simulink model "LunarMicrogrid_Combined_PVOnly_backup"  (R2026b)
settings: Solver=ode23t  StopTime=simulation.timeSim  MaxStep=1/(5*solarPlant.converterSwitchingFrequency)  AbsTol=1e-3
PreLoadFcn:
  | run('LunarMicrogridA_Data');
undefined symbols (not defined in the file or in its folder): battery, bms, bmsController, boostController, connectedLoad, dcVoltage, lunarCase, maxSoC, maxVdc, minIrrad, minSoC, minVdc, olTime, sensor, solarPanel, solarPlant
libraries: fl_lib x17, nesl_utility x15, simulink x13, ee_lib x6, eePwmGenerator x3, simulink_extras x2, batteryecm_lib x1
(part 1 of 2)
settings Model: Creator=The MathWorks, Inc.  LastModifiedBy=Samiya
settings SolverCC: AutoScaleAbsTol=off
settings DataIOCC: DSMLogging=off  ReturnWorkspaceOutputs=off  SaveOutput=off  SaveTime=off  SignalLoggingName=SolarPVDCWithBattery_logDB
settings OptimizationCC: ReuseModelBlockBuffer=off
settings DebuggingCC: SymbolicDimsDataTypeCodeGenerationDiagnostic=none
settings SFSimCC: CustomCodeUndefinedFunction=UseInterfaceOnly
settings RTWCC: DLArmComputeVersion=19.05
settings SimscapeCC: SimscapeLogName=simlog_SolarPVDCWithBattery  SimscapeLogSimulationStatistics=on  SimscapeLogType=all  SimscapeUseEnergyAccounting=off

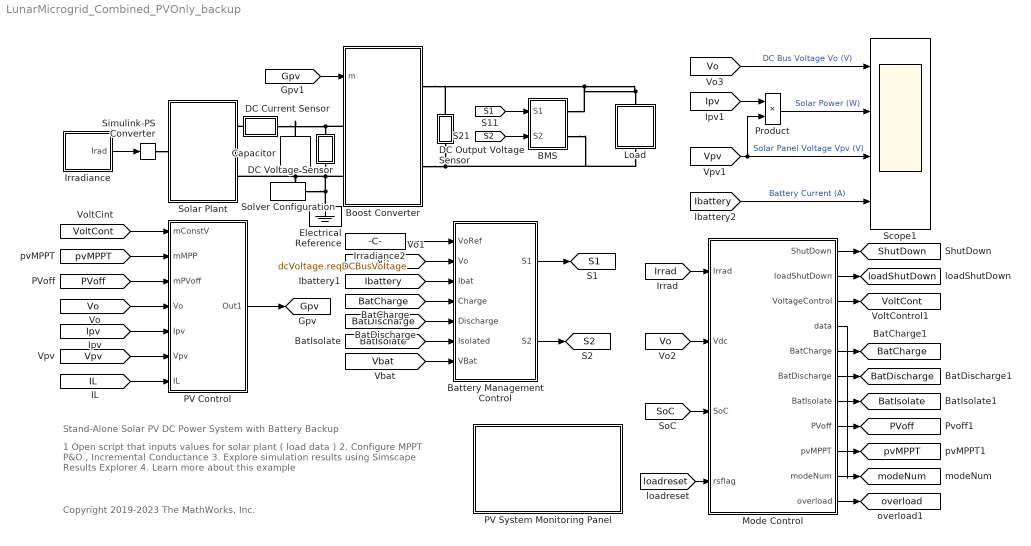
== system LunarMicrogrid_Combined_PVOnly_backup ==
  note: 1 Open script that inputs values for solar plant ( load data )
      | 2. Configure MPPT P&O , Incremental Conductance
      | 3. Explore simulation results using Simscape Results Explorer
      | 4. Learn more about this example
  note: Stand-Alone Solar PV DC Power System with Battery Backup
  note: Copyright 2019-2023 The MathWorks, Inc.
  BMS : Subsystem
  Battery Management Control : Subsystem
  Boost Converter : Subsystem  VariantControl=boostCircuit == 1
  Capacitor : fl_lib/Electrical/Electrical Elements/Capacitor  c=boost.inputCapacitor F  r=1e-6 Ohm  g=0 1/Ohm  i_specify=off  i_priority=None  i=0 A  i_nominal_specify=off  i_nominal_value=1  i_nominal_unit=A  v_specify=off  v_priority=None  v=solarPlant.startMPPTValue V  v_nominal_specify=off  v_nominal_value=1  v_nominal_unit=V  vc_specify=on  vc_priority=High  vc=solarPVInputCapacitorInitialVoltage V  vc_nominal_specify=off  vc_nominal_value=1  vc_nominal_unit=V
  DC Current Sensor : Subsystem
      mask Display: disp('i')
  DC Output Voltage Sensor : Subsystem
      mask Display: disp('v')
  DC Voltage Sensor : Subsystem
      mask Display: disp('v');
  Electrical Reference : fl_lib/Electrical/Electrical Elements/Electrical Reference
  Irradiance : Subsystem
  Irradiance2 : Constant  Value=dcVoltage.reqDCBusVoltage
  Load : Subsystem
  Mode Control : Stateflow chart  TreatAsAtomicUnit=on
  PV Control : Subsystem
  PV System Monitoring Panel : Subsystem
  Product : Product
  Scope1 : Scope  NumInputPorts=4
      settings: TimeSpan=simulation.timeSim  ActiveDisplayYMinimum=-72.27632  ActiveDisplayYMaximum=650.48692
  Simulink-PS Converter : nesl_utility/Simulink-PS Converter  PhysicalDomain=network_engine_domain  SubClassName=ps_input  LeftPortType=input  RightPortType=output  PseudoPeriodic=off  Frequencies=[]  NoiseDistribution=none  NoiseParameters=[]  Unit=1  AffineConversion=off  FilteringAndDerivatives=provide  SimscapeFilterOrder=1  InputFilterTimeConstant=0.001  UdotUserProvided=0
  Solar Plant : Subsystem
  Solver Configuration : nesl_utility/Solver Configuration  PhysicalDomain=network_engine_domain  SubClassName=solver  LeftPortType=input  RightPortType=generic  Tones=[]  Harmonics=[]  SimulateNoise=off  Profile=off  UseLocalSampling=off  EnableSwitchedLinearOptims=on  FrequencyDomain=off  UseCCode=off  RelTol=0.001  AbsTol=1e-06  MinStep=1e-09  ToWorkspace=off  RevertToSquareIcSolve=off  NumHomotopyIterations=100  PhasorMode=off  PhasorModeNumHarmonics=1  ConsistencySolver=NEWTON_FTOL  CanonicalOrdering=UNORDERED  OptimizeIntermediates=UNOPTIMIZED  MulticoreSolverChoice=BACKWARD_EULER  IndexReductionMethod=DerivativeReplacement  DoDC=off  ResidualTolerance=1e-9  ConsistencyTolSource=GLOBAL  ConsistencyAbsTol=0.001  ConsistencyRelTol=0.001  ConsistencyTolFactor=0.001  UseLocalSolver=off  LocalSolverChoice=NE_TRAPEZOIDAL_ADVANCER  ResolveIndetEquations=on  FunctionEvalNumThread=1  LocalSolverSampleTime=2e-6  DoFixedCost=off  MaxNonlinIter=10  MaxModeIter=2  ComputeImpulses=off  ImpulseIterations=2  LinearAlgebra=auto  LinearAlgebraNumThread=0  EquationFormulation=NE_TIME_EF  DelaysMemoryBudget=1024  AutomaticFiltering=on  FilteringTimeConstant=0.001  PartitionStorageMethod=AS_NEEDED  PartitionMemoryBudget=1024  PartitionMethod=FAST  MultibodyUseLocalSolver=off  MultibodyLocalSolverChoice=ODE1  MultibodyLocalSolverSampleTime=0.001
  tag scope: BatCharge=global, BatDischarge=global, BatIsolate=global, Gpv=global, PVoff=global, S1=global, S2=global, ShutDown=global, VoltCont=global, loadShutDown=global, modeNum=global, overload=global, pvMPPT=global
  wires:
  Mode Control/6(BatDischarge) -> [BatDischarge]
  [Vpv] -> Scope1/3, Product/2  "Solar Panel Voltage Vpv (V)"
  Battery Management Control/2(S2) -> [S2]
  [Ibattery] -> Battery Management Control/3(Ibat)
  Product/1 -> Scope1/2  "Solar Power (W)"
  [Vbat] -> Battery Management Control/7(VBat)
  [Ipv] -> PV Control/5(Ipv)
  Irradiance/1(Irad) -> Simulink-PS Converter/1
  [IL] -> PV Control/7(IL)
  Mode Control/2(loadShutDown) -> [loadShutDown]
  Mode Control/10(modeNum) -> [modeNum]
  [BatDischarge] -> Battery Management Control/5(Discharge)
  Mode Control/11(overload) -> [overload]
  [Ipv] -> Product/1
  [PVoff] -> PV Control/3(mPVoff)
  Mode Control/1(ShutDown) -> [ShutDown]
  Mode Control/3(VoltageControl) -> [VoltCont]
  [BatIsolate] -> Battery Management Control/6(Isolated)
  [Vo] -> Mode Control/2(Vdc)
  [pvMPPT] -> PV Control/2(mMPP)
  Mode Control/9(pvMPPT) -> [pvMPPT]
  [loadreset] -> Mode Control/4(rsflag)
  [SoC] -> Mode Control/3(SoC)
  Mode Control/7(BatIsolate) -> [BatIsolate]
  [Gpv] -> Boost Converter/1(m)
  PV Control/1(Out1) -> [Gpv]
  Irradiance2/1 -> Battery Management Control/1(VoRef)
  [VoltCont] -> PV Control/1(mConstV)
  [Irrad] -> Mode Control/1(Irrad)
  Mode Control/8(PVoff) -> [PVoff]
  [Vo] -> Scope1/1  "DC Bus Voltage Vo (V)"
  Mode Control/5(BatCharge) -> [BatCharge]
  Battery Management Control/1(S1) -> [S1]
  [Ibattery] -> Scope1/4  "Battery Current (A)"
  [Vo] -> PV Control/4(Vo)
  [Vo] -> Battery Management Control/2(Vo)
  [S2] -> BMS/2(S2)
  [Vpv] -> PV Control/6(Vpv)
  [BatCharge] -> Battery Management Control/4(Charge)
  [S1] -> BMS/1(S1)
  Mode Control/4(data) -> ?
  connections:
  Load/LConn1 -- BMS/RConn1 -- Boost Converter/RConn1 -- DC Output Voltage Sensor/RConn1
  Boost Converter/RConn2 -- BMS/RConn2 -- Load/RConn1 -- DC Output Voltage Sensor/LConn1
  Solver Configuration/RConn1 -- Solar Plant/RConn2 -- Capacitor/RConn1 -- Boost Converter/LConn2 -- DC Voltage Sensor/LConn1 -- Electrical Reference/LConn1
  Boost Converter/LConn1 -- DC Voltage Sensor/RConn1 -- DC Current Sensor/LConn1 -- Capacitor/LConn1
  DC Current Sensor/RConn1 -- Solar Plant/RConn1
  Simulink-PS Converter/RConn1 -- Solar Plant/LConn1

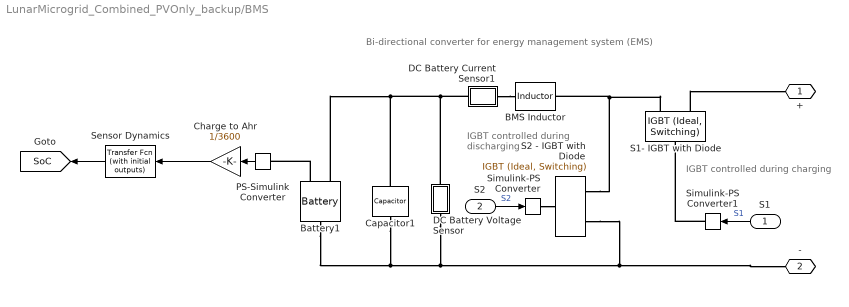
== system LunarMicrogrid_Combined_PVOnly_backup/BMS ==
  note: IGBT controlled during charging
  note: Bi-directional converter for energy management system (EMS)
  note: IGBT controlled during discharging
  S1 : Inport
  S2 : Inport  Port=2
  BMS Inductor : fl_lib/Electrical/Electrical Elements/Inductor  l=bms.batteryChargingInductor H  r=bms.batteryChargingInductorResistance Ohm  g=1e-9 1/Ohm  i_specify=off  i_priority=High  i=0 A  i_nominal_specify=off  i_nominal_value=1  i_nominal_unit=A  v_specify=off  v_priority=High  v=0 V  v_nominal_specify=off  v_nominal_value=1  v_nominal_unit=V  i_L_specify=on  i_L_priority=High  i_L=0 A  i_L_nominal_specify=off  i_L_nominal_value=1  i_L_nominal_unit=A
      settings: LogSimulationData=on
  Battery1 : batteryecm_lib/Battery  Vnom=battery.nominalBatteryVoltage V  prm_dir=1  R1_dis=2 Ohm  R1_ch=2 Ohm  R1=0.01 Ohm  prm_AH=2  AH=connectedLoad.batteryAmpHr hr*A  V1=battery.minBatteryNominalVoltage V  AH1=connectedLoad.batteryAmpHr*0.2 hr*A  prm_R2=2  R2=2000 Ohm  Tmeas=298.15 K  charge_measurement_port=simscape.enum.battery.enable.yes  prm_dyn=1  Rp1=0.005 Ohm  tau1=30 s  Rp2=0.005 Ohm  tau2=30 s  Rp3=0.005 Ohm  tau3=30 s  Rp4=0.005 Ohm  tau4=30 s  Rp5=0.005 Ohm  tau5=30 s  prm_fade=1  N_fade=100  AH_fade=45 hr*A  R1_fade=2.02 Ohm  R1_ch_fade=2.02 Ohm  V1_fade=10.35 V  prm_age=1  prm_age_OCV=1  OCV_age=0.9  SOC_age=60  Tmeas_age=298.15 K  delta_time_age_vec=[0] d  temperature_age_vec=[273] K  OCV_scaling_age=2.2134e6  OCV_offset_age=1.632e6  temp_exp_age=0.515833569 V  t_exp_age=0.75  Vnom_T2=12 V  R1_T2=2.2 Ohm  R1_T2_dis=2.2 Ohm  R1_T2_ch=2.2 Ohm  V1_T2=11.4 V  R2_T2=2200 Ohm  Rp1_T2=0.005 Ohm  tau1_T2=30 s  Rp2_T2=0.005 Ohm  tau2_T2=30 s  Rp3_T2=0.005 Ohm  tau3_T2=30 s  Rp4_T2=0.005 Ohm  tau4_T2=30 s  Rp5_T2=0.005 Ohm  tau5_T2=30 s  Tmeas2=273.15 K  thermal_port=simscape.enum.thermaleffects.omit  thermal_mass=30000 J/K  i_specify=off  i_priority=None  i=0 A  i_nominal_specify=off  i_nominal_value=1  i_nominal_unit=A  v_specify=off  v_priority=None  v=0 V  v_nominal_specify=off  v_nominal_value=1  v_nominal_unit=V  charge_specify=on  charge_priority=High  charge=batteryInitialStateOfCharge hr*A  charge_nominal_specify=off  charge_nominal_value=1  charge_nominal_unit=A*hr  num_cycles_specify=off  num_cycles_priority=High  num_cycles=0  num_cycles_nominal_specify=off  num_cycles_nominal_value=1  num_cycles_nominal_unit=1  temperature_specify=off  temperature_priority=High  temperature=298.15 K  temperature_nominal_specify=off  temperature_nominal_value=1  temperature_nominal_unit=K
  Capacitor1 : fl_lib/Electrical/Electrical Elements/Capacitor  c=boost.outputCapacitor F  r=1e-6 Ohm  g=0 1/Ohm  i_specify=off  i_priority=None  i=0 A  i_nominal_specify=off  i_nominal_value=1  i_nominal_unit=A  v_specify=off  v_priority=None  v=0 V  v_nominal_specify=off  v_nominal_value=1  v_nominal_unit=V  vc_specify=on  vc_priority=High  vc=batteryInputCapacitorInitialVoltage V  vc_nominal_specify=off  vc_nominal_value=1  vc_nominal_unit=V
  Charge to Ahr : Gain  Gain=1/3600
  DC Battery Current Sensor1 : Subsystem
      mask Display: disp('i');
  DC Battery Voltage Sensor : Subsystem
      mask Display: disp('v');
  PS-Simulink Converter : nesl_utility/PS-Simulink Converter  PhysicalDomain=network_engine_domain  SubClassName=ps_output  LeftPortType=input  RightPortType=output  PseudoPeriodic=off  Frequencies=[]  VectorFormat=1-D array  Unit=inherit  AffineConversion=off
  S1- IGBT with Diode : ee_lib/Semiconductors & Converters/IGBT (Ideal, Switching)  port_option=ee.enum.controlport.ps  Vf=0.1 V  Ron=0.001 Ohm  Goff=1e-5 1/Ohm  Vth=2.5 V  diode_param=2  diode_Vf=0.1 V  diode_Ron=0.001 Ohm  diode_Goff=1e-5 1/Ohm  diode_C=50e-9 F  diode_iRM=-235 A  diode_iF=300 A  diode_idot=-50 A/us  diode_trr_param=1  diode_trr_factor=3  diode_trr=15 us  diode_Qrr=1500 s*uA  ice_specify=off  ice_priority=None  ice=0 A  ice_nominal_specify=off  ice_nominal_value=1  ice_nominal_unit=A  vce_specify=off  vce_priority=None  vce=0 V  vce_nominal_specify=off  vce_nominal_value=1  vce_nominal_unit=V  vge_specify=off  vge_priority=None  vge=0 V  vge_nominal_specify=off  vge_nominal_value=1  vge_nominal_unit=V  thermal_loss_option=ee.enum.converters.thermalLossOption.constantvalues  Von_data=[0, .1, .6, .8, 1, 1.3, 1.6, 2, 2.4; 0, .1, .7, 1, 1.2, 1.5, 1.9, 2.4, 2.8] V  Tj=[298.15, 398.15] K  Iout_data=[0, .1, 1, 5, 10, 20, 40, 70, 100] A  tabulateWithVce=false  Eon_data=[0, .0024, .024, .12, .2, .48, 1.04, 2.16, 3.24; 0, .003, .03, .15, .25, .6, 1.3, 2.7, 4.05] * 1e-3 J  Eoff_data=[0, .0007, .0066, .033, .066, .17, .33, .83, 1.5; 0, .001, .01, .05, .1, .25, .5, 1.2, 2.2] * 1e-3 J  Eon_data_3D=[zeros(2, 9, 3)] J  Eoff_data_3D=[zeros(2, 9, 3)] J  Tj_loss=[298.15, 398.15] K  Iout_data_loss=[0, .1, 1, 5, 10, 20, 40, 70, 100] A  Vce_loss=[0, 150, 300] V  Eon_scalar=22.86e-3 J  Eoff_scalar=17.14e-3 J  Voff=300 V  Iout_scalar=600 A  useCurrentFromPreviousCycle=true  currentMeasDelay=0 s  useVoltageFromPreviousCycle=true  voltageMeasDelay=0 s  diodeModelType=ee.enum.converters.diodeModelType.pwl  diodeTableType=ee.enum.diode.tableType.IfMat  diode_ReverseIVType=ee.enum.diode.diodeReverseIV.constant  diode_IfMat=[.07, .12, .19, 1.75, 4.24, 7.32, 11.2; .16, .3, .72, 2.14, 4.02, 6.35, 9.12] A  diode_VfMat=[.9, 1.15, 1.25, 1.5, 1.75, 2.17, 2.6, 2.85; .58, .68, .75, 1.1, 1.38, 1.77, 2.27, 2.7] V  diode_TjVec=[25, 125] degC  diode_VfVec=[.5, .7, .9, 1.3, 1.7, 2.1, 2.5] V  diode_IfVec=[.1, .2, .5, 1, 2, 4, 7, 10] A  diode_IrMat=[1e-06, 2e-06, 5e-06, 1e-05, 2.5e-05, 5e-05, .0001; 2e-06, 5e-06, 1e-05, 4e-05, 8e-05, .0002, .0005] A  diode_VrMat=[10, 100, 200, 250, 300, 325, 350; 10, 70, 160, 220, 270, 300, 320] V  diode_VrVec=[10, 20, 40, 50, 70, 80, 100] V  diode_IrVec=[1e-06, 2e-06, 5e-06, 1e-05, 2e-05, 5e-05, .0001] A  diode_Vr=-600 V  diode_Ls=150 nH  diode_Erec=0.03 J  diode_rec_loss_model=ee.enum.diode.reverseRecoveryModelTabulateUpTo3D.fixed  diode_ErecVal=0 J  diode_scaleWithIandV=true  diode_ErecMat=zeros(2, 3) J  diodeErecMat3D=zeros(2, 3, 2) J  diode_TjrecVec=[298.15, 398.15] K  diode_IfrecVec=[.1, 1, 10] A  diodeVrecVec=[0, 100] V  diode_IrecVal=10 A  diode_VrecVal=10 V  diode_tFilter=1 / 1000 / 100 s  separateThermalPortForDiode=false  thermal_network_parameterization=ee.enum.thermalNetworkTopology.external  Rth=[.08, .5] K/W  Rth_Cauer=[.08, .1, .5] K/W  Rth_Foster=[.08, .14, .22, .16] K/W  thermal_mass_parameterization=ee.enum.thermalNetwork.timeconstant  thermal_mass=[.01, .5] J/K  thermal_mass_Cauer=[.01, .1, .5] J/K  thermal_mass_Foster=[.001, .005, .05, .5] J/K  thermal_time_constant=[.001, .2] s  thermal_time_constant_Cauer=[.001, .1, .2] s  thermal_time_constant_Foster=[7e-05, .0007, .01, .08] s  thermal_mass_initial_temperatures=[25, 25] degC  thermal_mass_initial_temperatures_Cauer=[25, 25, 25] degC  junction_thermal_mass=0.01 J/K  Tvec_initial_Foster=[25, 25, 25, 25] degC  RthDiode=[.03, .2] K/W  RthCauerDiode=[.03, .1, .2] K/W  RthFosterDiode=[.03, .2] K/W  thermalMassDiode=[3, 25] J/K  thermalMassCauerDiode=[3, 10, 25] J/K  thermalMassFosterDiode=[33, 50] J/K  thermalTauDiode=[.1, 5] s  thermalTauCauerDiode=[.1, 1, 5] s  thermalTauFosterDiode=[1, 10] s  thermalMassInitTempDiode=[25, 25] degC  thermalMassInitTempCauerDiode=[25, 25, 25] degC  junctionthermalMassDiode=0.1 J/K  TVecInitialFosterDiode=[25, 25] degC  no_thermal_network=0  IGBT_junction_temperature_specify=off  IGBT_junction_temperature_priority=None  IGBT_junction_temperature=25 degC  IGBT_junction_temperature_nominal_specify=off  IGBT_junction_temperature_nominal_value=1  IGBT_junction_temperature_nominal_unit=degC  diode_junction_temperature_specify=off  diode_junction_temperature_priority=None  diode_junction_temperature=25 degC  diode_junction_temperature_nominal_specify=off  diode_junction_temperature_nominal_value=1  diode_junction_temperature_nominal_unit=degC  Qj_specify=off  Qj_priority=None  Qj=0 W  Qj_nominal_specify=off  Qj_nominal_value=1  Qj_nominal_unit=W  accumulatedSwitchingLosses_specify=off  accumulatedSwitchingLosses_priority=None  accumulatedSwitchingLosses=0 J
  S2 - IGBT with Diode : ee_lib/Semiconductors & Converters/IGBT (Ideal, Switching)  port_option=ee.enum.controlport.ps  Vf=0.1 V  Ron=0.001 Ohm  Goff=1e-5 1/Ohm  Vth=2.5 V  diode_param=2  diode_Vf=0.1 V  diode_Ron=0.001 Ohm  diode_Goff=1e-5 1/Ohm  diode_C=50e-9 F  diode_iRM=-235 A  diode_iF=300 A  diode_idot=-50 A/us  diode_trr_param=1  diode_trr_factor=3  diode_trr=15 us  diode_Qrr=1500 s*uA  ice_specify=off  ice_priority=None  ice=0 A  ice_nominal_specify=off  ice_nominal_value=1  ice_nominal_unit=A  vce_specify=off  vce_priority=None  vce=0 V  vce_nominal_specify=off  vce_nominal_value=1  vce_nominal_unit=V  vge_specify=off  vge_priority=None  vge=0 V  vge_nominal_specify=off  vge_nominal_value=1  vge_nominal_unit=V  thermal_loss_option=ee.enum.converters.thermalLossOption.constantvalues  Von_data=[0, .1, .6, .8, 1, 1.3, 1.6, 2, 2.4; 0, .1, .7, 1, 1.2, 1.5, 1.9, 2.4, 2.8] V  Tj=[298.15, 398.15] K  Iout_data=[0, .1, 1, 5, 10, 20, 40, 70, 100] A  tabulateWithVce=false  Eon_data=[0, .0024, .024, .12, .2, .48, 1.04, 2.16, 3.24; 0, .003, .03, .15, .25, .6, 1.3, 2.7, 4.05] * 1e-3 J  Eoff_data=[0, .0007, .0066, .033, .066, .17, .33, .83, 1.5; 0, .001, .01, .05, .1, .25, .5, 1.2, 2.2] * 1e-3 J  Eon_data_3D=[zeros(2, 9, 3)] J  Eoff_data_3D=[zeros(2, 9, 3)] J  Tj_loss=[298.15, 398.15] K  Iout_data_loss=[0, .1, 1, 5, 10, 20, 40, 70, 100] A  Vce_loss=[0, 150, 300] V  Eon_scalar=22.86e-3 J  Eoff_scalar=17.14e-3 J  Voff=300 V  Iout_scalar=600 A  useCurrentFromPreviousCycle=true  currentMeasDelay=0 s  useVoltageFromPreviousCycle=true  voltageMeasDelay=0 s  diodeModelType=ee.enum.converters.diodeModelType.pwl  diodeTableType=ee.enum.diode.tableType.IfMat  diode_ReverseIVType=ee.enum.diode.diodeReverseIV.constant  diode_IfMat=[.07, .12, .19, 1.75, 4.24, 7.32, 11.2; .16, .3, .72, 2.14, 4.02, 6.35, 9.12] A  diode_VfMat=[.9, 1.15, 1.25, 1.5, 1.75, 2.17, 2.6, 2.85; .58, .68, .75, 1.1, 1.38, 1.77, 2.27, 2.7] V  diode_TjVec=[25, 125] degC  diode_VfVec=[.5, .7, .9, 1.3, 1.7, 2.1, 2.5] V  diode_IfVec=[.1, .2, .5, 1, 2, 4, 7, 10] A  diode_IrMat=[1e-06, 2e-06, 5e-06, 1e-05, 2.5e-05, 5e-05, .0001; 2e-06, 5e-06, 1e-05, 4e-05, 8e-05, .0002, .0005] A  diode_VrMat=[10, 100, 200, 250, 300, 325, 350; 10, 70, 160, 220, 270, 300, 320] V  diode_VrVec=[10, 20, 40, 50, 70, 80, 100] V  diode_IrVec=[1e-06, 2e-06, 5e-06, 1e-05, 2e-05, 5e-05, .0001] A  diode_Vr=-600 V  diode_Ls=150 nH  diode_Erec=0.03 J  diode_rec_loss_model=ee.enum.diode.reverseRecoveryModelTabulateUpTo3D.fixed  diode_ErecVal=0 J  diode_scaleWithIandV=true  diode_ErecMat=zeros(2, 3) J  diodeErecMat3D=zeros(2, 3, 2) J  diode_TjrecVec=[298.15, 398.15] K  diode_IfrecVec=[.1, 1, 10] A  diodeVrecVec=[0, 100] V  diode_IrecVal=10 A  diode_VrecVal=10 V  diode_tFilter=1 / 1000 / 100 s  separateThermalPortForDiode=false  thermal_network_parameterization=ee.enum.thermalNetworkTopology.external  Rth=[.08, .5] K/W  Rth_Cauer=[.08, .1, .5] K/W  Rth_Foster=[.08, .14, .22, .16] K/W  thermal_mass_parameterization=ee.enum.thermalNetwork.timeconstant  thermal_mass=[.01, .5] J/K  thermal_mass_Cauer=[.01, .1, .5] J/K  thermal_mass_Foster=[.001, .005, .05, .5] J/K  thermal_time_constant=[.001, .2] s  thermal_time_constant_Cauer=[.001, .1, .2] s  thermal_time_constant_Foster=[7e-05, .0007, .01, .08] s  thermal_mass_initial_temperatures=[25, 25] degC  thermal_mass_initial_temperatures_Cauer=[25, 25, 25] degC  junction_thermal_mass=0.01 J/K  Tvec_initial_Foster=[25, 25, 25, 25] degC  RthDiode=[.03, .2] K/W  RthCauerDiode=[.03, .1, .2] K/W  RthFosterDiode=[.03, .2] K/W  thermalMassDiode=[3, 25] J/K  thermalMassCauerDiode=[3, 10, 25] J/K  thermalMassFosterDiode=[33, 50] J/K  thermalTauDiode=[.1, 5] s  thermalTauCauerDiode=[.1, 1, 5] s  thermalTauFosterDiode=[1, 10] s  thermalMassInitTempDiode=[25, 25] degC  thermalMassInitTempCauerDiode=[25, 25, 25] degC  junctionthermalMassDiode=0.1 J/K  TVecInitialFosterDiode=[25, 25] degC  no_thermal_network=0  IGBT_junction_temperature_specify=off  IGBT_junction_temperature_priority=None  IGBT_junction_temperature=25 degC  IGBT_junction_temperature_nominal_specify=off  IGBT_junction_temperature_nominal_value=1  IGBT_junction_temperature_nominal_unit=degC  diode_junction_temperature_specify=off  diode_junction_temperature_priority=None  diode_junction_temperature=25 degC  diode_junction_temperature_nominal_specify=off  diode_junction_temperature_nominal_value=1  diode_junction_temperature_nominal_unit=degC  Qj_specify=off  Qj_priority=None  Qj=0 W  Qj_nominal_specify=off  Qj_nominal_value=1  Qj_nominal_unit=W  accumulatedSwitchingLosses_specify=off  accumulatedSwitchingLosses_priority=None  accumulatedSwitchingLosses=0 J
  Sensor Dynamics : simulink_extras/Additional Linear/Transfer Fcn (with initial outputs)  N=[1]  D=[1/sensor.samplingFreq 1]  Y0=minSoC  U0=0
  Simulink-PS Converter : nesl_utility/Simulink-PS Converter  PhysicalDomain=network_engine_domain  SubClassName=ps_input  LeftPortType=input  RightPortType=output  PseudoPeriodic=off  Frequencies=[]  NoiseDistribution=none  NoiseParameters=[]  Unit=1  AffineConversion=off  FilteringAndDerivatives=provide  SimscapeFilterOrder=1  InputFilterTimeConstant=0.001  UdotUserProvided=0
  Simulink-PS Converter1 : nesl_utility/Simulink-PS Converter  PhysicalDomain=network_engine_domain  SubClassName=ps_input  LeftPortType=input  RightPortType=output  PseudoPeriodic=off  Frequencies=[]  NoiseDistribution=none  NoiseParameters=[]  Unit=1  AffineConversion=off  FilteringAndDerivatives=provide  SimscapeFilterOrder=1  InputFilterTimeConstant=0.001  UdotUserProvided=0
  + : PMIOPort  Side=Right
  - : PMIOPort  Port=2  Side=Right
  tag scope: SoC=global
  wires:
  S2/1 -> Simulink-PS Converter/1  "S2"
  S1/1 -> Simulink-PS Converter1/1  "S1"
  PS-Simulink Converter/1 -> Charge to Ahr/1
  Sensor Dynamics/1 -> [SoC]
  Charge to Ahr/1 -> Sensor Dynamics/1
  connections:
  S2 - IGBT with Diode/RConn2 -- Battery1/RConn1 -- Capacitor1/RConn1 -- DC Battery Voltage Sensor/LConn1 -- -/RConn1
  S2 - IGBT with Diode/RConn1 -- S1- IGBT with Diode/RConn2 -- BMS Inductor/RConn1
  S1- IGBT with Diode/RConn1 -- +/RConn1
  Simulink-PS Converter/RConn1 -- S2 - IGBT with Diode/LConn1
  Battery1/LConn2 -- PS-Simulink Converter/LConn1
  Simulink-PS Converter1/RConn1 -- S1- IGBT with Diode/LConn1
  DC Battery Current Sensor1/RConn1 -- BMS Inductor/LConn1
  DC Battery Current Sensor1/LConn1 -- DC Battery Voltage Sensor/RConn1 -- Battery1/LConn1 -- Capacitor1/LConn1

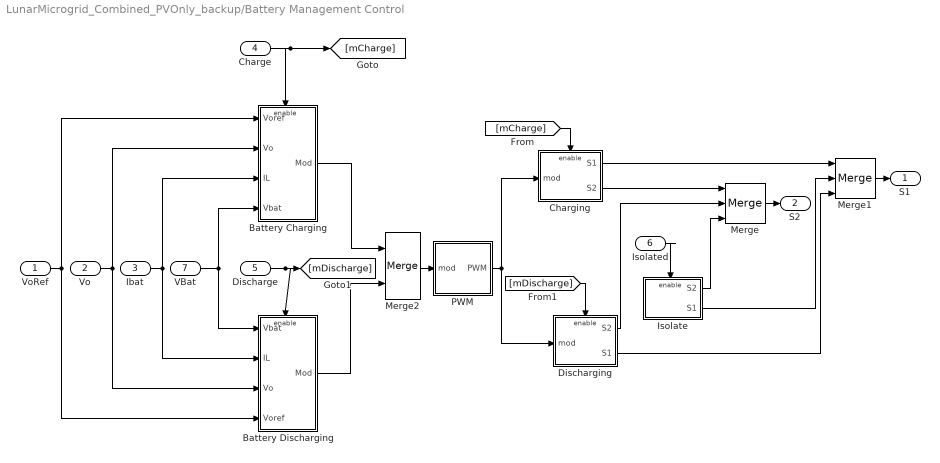
== system LunarMicrogrid_Combined_PVOnly_backup/Battery Management Control ==
  VoRef : Inport
  Vo : Inport  Port=2
  Ibat : Inport  Port=3
  Charge : Inport  Port=4
  Discharge : Inport  Port=5
  Isolated : Inport  Port=6
  VBat : Inport  Port=7
  Battery Charging : Subsystem
  Battery Discharging : Subsystem
  Charging : Subsystem  TreatAsAtomicUnit=on
  Discharging : Subsystem  TreatAsAtomicUnit=on
  Isolate : Subsystem  TreatAsAtomicUnit=on
  Merge : Merge  Inputs=3
  Merge1 : Merge  Inputs=3
  Merge2 : Merge
  PWM : Subsystem
  S1 : Outport
  S2 : Outport  Port=2
  wires:
  Charging/2(S2) -> Merge/1
  Discharging/1(S2) -> Merge/2
  Charging/1(S1) -> Merge1/1
  Isolate/1(S2) -> Merge/3
  Isolate/2(S1) -> Merge1/2
  Discharging/2(S1) -> Merge1/3
  Merge1/1 -> S1/1
  Isolated/1 -> Isolate/Enable
  Vo/1 -> Battery Charging/2(Vo), Battery Discharging/3(Vo)
  Ibat/1 -> Battery Charging/3(IL), Battery Discharging/2(IL)
  Battery Charging/1(Mod) -> Merge2/1
  Battery Discharging/1(Mod) -> Merge2/2
  Merge/1 -> S2/1
  Charge/1 -> [mCharge], Battery Charging/Enable
  Discharge/1 -> Battery Discharging/Enable, [mDischarge]
  [mCharge] -> Charging/Enable
  [mDischarge] -> Discharging/Enable
  PWM/1(PWM) -> Charging/1(mod), Discharging/1(mod)
  Merge2/1 -> PWM/1(mod)
  VoRef/1 -> Battery Charging/1(Voref), Battery Discharging/4(Voref)
  VBat/1 -> Battery Discharging/1(Vbat), Battery Charging/4(Vbat)

== system LunarMicrogrid_Combined_PVOnly_backup/Boost Converter ==
  m : Inport
  AC Current Sensor1 : Subsystem
      mask Display: disp('i');
  DC Bus Capacitor : fl_lib/Electrical/Electrical Elements/Capacitor  c=boost.outputCapacitor F  r=1e-6 Ohm  g=0 1/Ohm  i_specify=off  i_priority=None  i=0 A  i_nominal_specify=off  i_nominal_value=1  i_nominal_unit=A  v_specify=off  v_priority=None  v=0 V  v_nominal_specify=off  v_nominal_value=1  v_nominal_unit=V  vc_specify=on  vc_priority=High  vc=boostOutputCapacitorInitialVoltage V  vc_nominal_specify=off  vc_nominal_value=1  vc_nominal_unit=V
  Diode : fl_lib/Electrical/Electrical Elements/Diode  Vf=0.6 V  Ron=0.3 Ohm  Goff=1e-8 1/Ohm  i_specify=off  i_priority=None  i=0 A  i_nominal_specify=off  i_nominal_value=1  i_nominal_unit=A  v_specify=off  v_priority=None  v=0 V  v_nominal_specify=off  v_nominal_value=1  v_nominal_unit=V
  Gain : Gain  Gain=5
  "IGBT (Ideal, Switching)" : ee_lib/Semiconductors & Converters/IGBT (Ideal, Switching)  port_option=ee.enum.controlport.ps  Vf=0.8 V  Ron=0.001 Ohm  Goff=1e-5 1/Ohm  Vth=2.5 V  diode_param=1  diode_Vf=0.8 V  diode_Ron=0.001 Ohm  diode_Goff=1e-5 1/Ohm  diode_C=50e-9 F  diode_iRM=-235 A  diode_iF=300 A  diode_idot=-50 A/us  diode_trr_param=1  diode_trr_factor=3  diode_trr=15 us  diode_Qrr=1500 s*uA  ice_specify=off  ice_priority=None  ice=0 A  ice_nominal_specify=off  ice_nominal_value=1  ice_nominal_unit=A  vce_specify=off  vce_priority=None  vce=0 V  vce_nominal_specify=off  vce_nominal_value=1  vce_nominal_unit=V  vge_specify=off  vge_priority=None  vge=0 V  vge_nominal_specify=off  vge_nominal_value=1  vge_nominal_unit=V  thermal_loss_option=ee.enum.converters.thermalLossOption.constantvalues  Von_data=[0, .1, .6, .8, 1, 1.3, 1.6, 2, 2.4; 0, .1, .7, 1, 1.2, 1.5, 1.9, 2.4, 2.8] V  Tj=[298.15, 398.15] K  Iout_data=[0, .1, 1, 5, 10, 20, 40, 70, 100] A  tabulateWithVce=false  Eon_data=[0, .0024, .024, .12, .2, .48, 1.04, 2.16, 3.24; 0, .003, .03, .15, .25, .6, 1.3, 2.7, 4.05] * 1e-3 J  Eoff_data=[0, .0007, .0066, .033, .066, .17, .33, .83, 1.5; 0, .001, .01, .05, .1, .25, .5, 1.2, 2.2] * 1e-3 J  Eon_data_3D=[zeros(2, 9, 3)] J  Eoff_data_3D=[zeros(2, 9, 3)] J  Tj_loss=[298.15, 398.15] K  Iout_data_loss=[0, .1, 1, 5, 10, 20, 40, 70, 100] A  Vce_loss=[0, 150, 300] V  Eon_scalar=22.86e-3 J  Eoff_scalar=17.14e-3 J  Voff=300 V  Iout_scalar=600 A  useCurrentFromPreviousCycle=true  currentMeasDelay=0 s  useVoltageFromPreviousCycle=true  voltageMeasDelay=0 s  diodeModelType=ee.enum.converters.diodeModelType.pwl  diodeTableType=ee.enum.diode.tableType.IfMat  diode_ReverseIVType=ee.enum.diode.diodeReverseIV.constant  diode_IfMat=[.07, .12, .19, 1.75, 4.24, 7.32, 11.2; .16, .3, .72, 2.14, 4.02, 6.35, 9.12] A  diode_VfMat=[.9, 1.15, 1.25, 1.5, 1.75, 2.17, 2.6, 2.85; .58, .68, .75, 1.1, 1.38, 1.77, 2.27, 2.7] V  diode_TjVec=[25, 125] degC  diode_VfVec=[.5, .7, .9, 1.3, 1.7, 2.1, 2.5] V  diode_IfVec=[.1, .2, .5, 1, 2, 4, 7, 10] A  diode_IrMat=[1e-06, 2e-06, 5e-06, 1e-05, 2.5e-05, 5e-05, .0001; 2e-06, 5e-06, 1e-05, 4e-05, 8e-05, .0002, .0005] A  diode_VrMat=[10, 100, 200, 250, 300, 325, 350; 10, 70, 160, 220, 270, 300, 320] V  diode_VrVec=[10, 20, 40, 50, 70, 80, 100] V  diode_IrVec=[1e-06, 2e-06, 5e-06, 1e-05, 2e-05, 5e-05, .0001] A  diode_Vr=-600 V  diode_Ls=150 nH  diode_Erec=0.03 J  diode_rec_loss_model=ee.enum.diode.reverseRecoveryModelTabulateUpTo3D.fixed  diode_ErecVal=0 J  diode_scaleWithIandV=true  diode_ErecMat=zeros(2, 3) J  diodeErecMat3D=zeros(2, 3, 2) J  diode_TjrecVec=[298.15, 398.15] K  diode_IfrecVec=[.1, 1, 10] A  diodeVrecVec=[0, 100] V  diode_IrecVal=10 A  diode_VrecVal=10 V  diode_tFilter=1 / 1000 / 100 s  separateThermalPortForDiode=false  thermal_network_parameterization=ee.enum.thermalNetworkTopology.external  Rth=[.08, .5] K/W  Rth_Cauer=[.08, .1, .5] K/W  Rth_Foster=[.08, .14, .22, .16] K/W  thermal_mass_parameterization=ee.enum.thermalNetwork.timeconstant  thermal_mass=[.01, .5] J/K  thermal_mass_Cauer=[.01, .1, .5] J/K  thermal_mass_Foster=[.001, .005, .05, .5] J/K  thermal_time_constant=[.001, .2] s  thermal_time_constant_Cauer=[.001, .1, .2] s  thermal_time_constant_Foster=[7e-05, .0007, .01, .08] s  thermal_mass_initial_temperatures=[25, 25] degC  thermal_mass_initial_temperatures_Cauer=[25, 25, 25] degC  junction_thermal_mass=0.01 J/K  Tvec_initial_Foster=[25, 25, 25, 25] degC  RthDiode=[.03, .2] K/W  RthCauerDiode=[.03, .1, .2] K/W  RthFosterDiode=[.03, .2] K/W  thermalMassDiode=[3, 25] J/K  thermalMassCauerDiode=[3, 10, 25] J/K  thermalMassFosterDiode=[33, 50] J/K  thermalTauDiode=[.1, 5] s  thermalTauCauerDiode=[.1, 1, 5] s  thermalTauFosterDiode=[1, 10] s  thermalMassInitTempDiode=[25, 25] degC  thermalMassInitTempCauerDiode=[25, 25, 25] degC  junctionthermalMassDiode=0.1 J/K  TVecInitialFosterDiode=[25, 25] degC  no_thermal_network=0  IGBT_junction_temperature_specify=off  IGBT_junction_temperature_priority=None  IGBT_junction_temperature=25 degC  IGBT_junction_temperature_nominal_specify=off  IGBT_junction_temperature_nominal_value=1  IGBT_junction_temperature_nominal_unit=degC  diode_junction_temperature_specify=off  diode_junction_temperature_priority=None  diode_junction_temperature=25 degC  diode_junction_temperature_nominal_specify=off  diode_junction_temperature_nominal_value=1  diode_junction_temperature_nominal_unit=degC  Qj_specify=off  Qj_priority=None  Qj=0 W  Qj_nominal_specify=off  Qj_nominal_value=1  Qj_nominal_unit=W  accumulatedSwitchingLosses_specify=off  accumulatedSwitchingLosses_priority=None  accumulatedSwitchingLosses=0 J
  MPPT Inductor : ee_lib/Passive/Inductor  l=boost.inductor H  enable_L_tol=0  L_tol=5  tol_distribution=1  nSigma=4  r=boost.inductorResistance Ohm  g=1e-9 1/Ohm  enable_operating_limits=0  operating_limit_action=2  max_working_current=1 A  power_rating=1 W  i_L_specify=on  i_L_priority=High  i_L=0 A  i_L_nominal_specify=off  i_L_nominal_value=1  i_L_nominal_unit=A
  Simulink-PS Converter : nesl_utility/Simulink-PS Converter  PhysicalDomain=network_engine_domain  SubClassName=ps_input  LeftPortType=input  RightPortType=output  PseudoPeriodic=off  Frequencies=[]  NoiseDistribution=none  NoiseParameters=[]  Unit=1  AffineConversion=off  FilteringAndDerivatives=provide  SimscapeFilterOrder=1  InputFilterTimeConstant=0.001  UdotUserProvided=0
  + : PMIOPort  Side=Left
  P : PMIOPort  Port=2  Side=Right
  N : PMIOPort  Port=3  Side=Right
  - : PMIOPort  Port=4  Side=Left
  wires:
  m/1 -> Gain/1
  Gain/1 -> Simulink-PS Converter/1
  connections:
  MPPT Inductor/LConn1 -- AC Current Sensor1/LConn1
  "IGBT (Ideal, Switching)"/RConn2 -- N/RConn1 -- DC Bus Capacitor/RConn1 -- -/RConn1
  AC Current Sensor1/RConn1 -- +/RConn1
  "IGBT (Ideal, Switching)"/LConn1 -- Simulink-PS Converter/RConn1
  MPPT Inductor/RConn1 -- "IGBT (Ideal, Switching)"/RConn1 -- Diode/LConn1
  DC Bus Capacitor/LConn1 -- Diode/RConn1 -- P/RConn1

== system LunarMicrogrid_Combined_PVOnly_backup/DC Current Sensor ==
  Current Sensor : fl_lib/Electrical/Electrical Sensors/Current Sensor
      settings: LogSimulationData=on
  PS-Simulink Converter : nesl_utility/PS-Simulink Converter  PhysicalDomain=network_engine_domain  SubClassName=ps_output  LeftPortType=input  RightPortType=output  PseudoPeriodic=off  Frequencies=[]  VectorFormat=1-D array  Unit=1  AffineConversion=off
  Sensor dynamics : TransferFcn  Numerator=1  Denominator=[1/sensor.samplingFreq 1]
  - : PMIOPort  Side=Left
  + : PMIOPort  Port=2  Side=Right
  tag scope: Ipv=global
  wires:
  PS-Simulink Converter/1 -> Sensor dynamics/1
  Sensor dynamics/1 -> [Ipv]
  connections:
  Current Sensor/RConn2 -- -/RConn1
  +/RConn1 -- Current Sensor/LConn1
  Current Sensor/RConn1 -- PS-Simulink Converter/LConn1

== system LunarMicrogrid_Combined_PVOnly_backup/DC Output Voltage Sensor ==
  PS-Simulink Converter : nesl_utility/PS-Simulink Converter  PhysicalDomain=network_engine_domain  SubClassName=ps_output  LeftPortType=input  RightPortType=output  PseudoPeriodic=off  Frequencies=[]  VectorFormat=1-D array  Unit=1  AffineConversion=off
  Sensor dynamics : TransferFcn  Numerator=1  Denominator=[1/sensor.samplingFreq 1]
  Voltage Sensor : fl_lib/Electrical/Electrical Sensors/Voltage Sensor
  - : PMIOPort  Side=Left
  + : PMIOPort  Port=2  Side=Right
  tag scope: Vo=global
  wires:
  PS-Simulink Converter/1 -> Sensor dynamics/1
  Sensor dynamics/1 -> [Vo]
  connections:
  Voltage Sensor/RConn2 -- -/RConn1
  Voltage Sensor/RConn1 -- PS-Simulink Converter/LConn1
  Voltage Sensor/LConn1 -- +/RConn1

== system LunarMicrogrid_Combined_PVOnly_backup/DC Voltage Sensor ==
  PS-Simulink Converter : nesl_utility/PS-Simulink Converter  PhysicalDomain=network_engine_domain  SubClassName=ps_output  LeftPortType=input  RightPortType=output  PseudoPeriodic=off  Frequencies=[]  VectorFormat=1-D array  Unit=1  AffineConversion=off
  Sensor dynamics : TransferFcn  Numerator=1  Denominator=[1/sensor.samplingFreq 1]
  Voltage Sensor : fl_lib/Electrical/Electrical Sensors/Voltage Sensor
      settings: LogSimulationData=on
  - : PMIOPort  Side=Left
  + : PMIOPort  Port=2  Side=Right
  tag scope: Vpv=global
  wires:
  PS-Simulink Converter/1 -> Sensor dynamics/1
  Sensor dynamics/1 -> [Vpv]
  connections:
  Voltage Sensor/LConn1 -- +/RConn1
  Voltage Sensor/RConn1 -- PS-Simulink Converter/LConn1
  Voltage Sensor/RConn2 -- -/RConn1

== system LunarMicrogrid_Combined_PVOnly_backup/Irradiance ==
  " " : Constant
  Sensor dynamics : TransferFcn  Numerator=1  Denominator=[1/sensor.samplingFreq 1]
  Solar Irradiance W/m2 : Gain  Gain=lunarCase.G_Wm2
  Irad : Outport
  tag scope: Irrad=global
  wires:
  " "/1 -> Solar Irradiance W/m2/1
  Solar Irradiance W/m2/1 -> Irad/1, Sensor dynamics/1
  Sensor dynamics/1 -> [Irrad]

== system LunarMicrogrid_Combined_PVOnly_backup/Load ==
  AC Current Sensor2 : Subsystem
      mask Display: disp('i');
  Load : Subsystem
  Load Flag : Subsystem
  Load Resistance : fl_lib/Electrical/Electrical Elements/Variable Resistor  Rmin=0 Ohm  thermalEnable=false  thermal_mass=1 J/K  i_specify=off  i_priority=None  i=5 A  i_nominal_specify=off  i_nominal_value=1  i_nominal_unit=A  v_specify=off  v_priority=None  v=0 V  v_nominal_specify=off  v_nominal_value=1  v_nominal_unit=V  T_specify=off  T_priority=None  T=300 K  T_nominal_specify=off  T_nominal_value=1  T_nominal_unit=K
  SPST Switch : ee_lib/Switches & Breakers/SPST Switch  R_closed=0.01 Ohm  G_open=1e-6 S  Threshold=0.5 V  Width=0 V  model_dynamics=0  t_on=1e-3 s  t_off=1e-3 s  initial_vT=0 V
  + : PMIOPort  Side=Left
  - : PMIOPort  Port=2  Side=Right
  connections:
  +/RConn1 -- SPST Switch/LConn2
  Load Resistance/LConn2 -- AC Current Sensor2/LConn1
  Load Resistance/RConn1 -- -/RConn1
  Load/RConn1 -- Load Resistance/LConn1
  Load Flag/RConn1 -- SPST Switch/LConn1
  AC Current Sensor2/RConn1 -- SPST Switch/RConn1

== system LunarMicrogrid_Combined_PVOnly_backup/PV Control ==
  mConstV : Inport
  mMPP : Inport  Port=2
  mPVoff : Inport  Port=3
  Vo : Inport  Port=4
  Ipv : Inport  Port=5
  Vpv : Inport  Port=6
  IL : Inport  Port=7
  Constant : Constant  Value=dcVoltage.reqDCBusVoltage
  Constant Voltage : Subsystem
  Maximum Power Point : Subsystem
  Merge : Merge  Inputs=3
  PV Isolate : Subsystem  TreatAsAtomicUnit=on
  Terminator : Terminator
  Out1 : Outport
  wires:
  Merge/1 -> Out1/1
  Vo/1 -> Maximum Power Point/2("Vo "), Constant Voltage/3("Vo ")
  PV Isolate/1(Gmpp) -> Merge/3
  Maximum Power Point/1(Gmpp) -> Merge/2
  mMPP/1 -> Maximum Power Point/Enable
  mConstV/1 -> Constant Voltage/Enable
  mPVoff/1 -> PV Isolate/Enable
  IL/1 -> Maximum Power Point/1("IL "), Constant Voltage/4(IL)
  Vpv/1 -> Maximum Power Point/3(Vpv), Constant Voltage/2(Vpv)
  Ipv/1 -> Maximum Power Point/4(Ipv)
  Constant/1 -> Constant Voltage/1(Vconst)
  Constant Voltage/1(G) -> Merge/1
  Maximum Power Point/2(Vmpp) -> Terminator/1

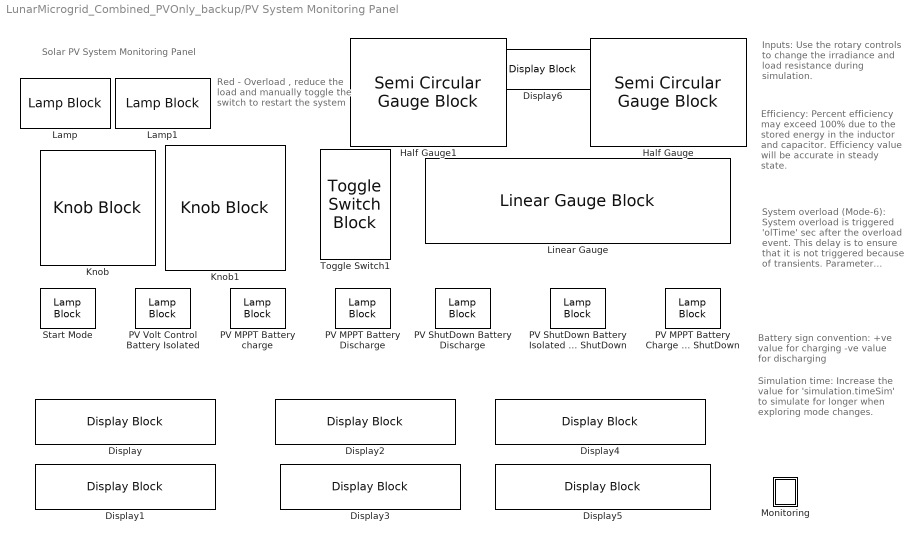
== system LunarMicrogrid_Combined_PVOnly_backup/PV System Monitoring Panel ==
  note: Red - Overload , reduce the load and manually toggle the switch to restart the system
  note: Solar PV System Monitoring Panel
  note: Simulation time:
      | Increase the value for 'simulation.timeSim' to simulate for longer when exploring mode changes.
  note: Inputs:
      | Use the rotary controls to change the irradiance and load resistance during simulation.
  note: System overload (Mode-6):
      | System overload is triggered 'olTime' sec after the overload event. This delay is to ensure that it is not triggered because of transients. Parameter 'olTime' can be modified in the supporting livescript.
  note: Efficiency:
      | Percent efficiency may exceed 100% due to the stored energy in the inductor and capacitor. Efficiency value will be accurate in steady state.
  note: Battery sign convention:
      | +ve value for charging
      | -ve value for discharging
  Display{,1..6} (7 alike) : DisplayBlock  Transparency=1  GridColor=[0.502, 0.502, 0.502]
  Half Gauge : SemiCircularGaugeBlock  ScaleMin=20  FontColor=[0.0, 0.0, 0.0]
  Half Gauge1 : SemiCircularGaugeBlock  FontColor=[0.0, 0.0, 0.0]
  Knob : KnobBlock  ScaleMin=150  ScaleMax=1000
  Knob1 : KnobBlock  ScaleMin=0.15  ScaleMax=20
  Lamp : LampBlock  DefaultColor=[192.0, 192.0, 192.0]
  Lamp1 : LampBlock  DefaultColor=[192.0, 192.0, 192.0]
  Linear Gauge : LinearGaugeBlock  ScaleMin=-100  FontColor=[0.0, 0.0, 0.0]
  Monitoring : Subsystem
  PV MPPT Battery Charge Load ShutDown : LampBlock  DefaultColor=[192.0, 192.0, 192.0]
  PV MPPT Battery Discharge : LampBlock  DefaultColor=[192.0, 192.0, 192.0]
  PV MPPT Battery charge : LampBlock  DefaultColor=[192.0, 192.0, 192.0]
  PV ShutDown Battery Discharge : LampBlock  DefaultColor=[192.0, 192.0, 192.0]
  PV ShutDown Battery Isolated System ShutDown : LampBlock  DefaultColor=[192.0, 192.0, 192.0]
  PV Volt Control Battery Isolated : LampBlock  DefaultColor=[192.0, 192.0, 192.0]
  Start Mode : LampBlock  DefaultColor=[192.0, 192.0, 192.0]
  Toggle Switch1 : ToggleSwitchBlock

== system LunarMicrogrid_Combined_PVOnly_backup/Solar Plant ==
  Current-Controlled Current Source- Scale panel current to Np parallel strings : fl_lib/Electrical/Electrical Sources/Current-Controlled Current Source  K=-1*(solarPlant.numParallelPanel-1)  i1_specify=off  i1_priority=None  i1=0 A  i1_nominal_specify=off  i1_nominal_value=1  i1_nominal_unit=A  i2_specify=off  i2_priority=None  i2=0 A  i2_nominal_specify=off  i2_nominal_value=1  i2_nominal_unit=A
  Solar Panel : Subsystem  mask(Solar Panel){}
      mask help: Models a solar panel using a parallel-connected sting of solar cells. The solar cell strings are modeled using a single Solar Cell block from the Simscape(TM) Electrical(TM) Sources library.
      mask Display: image('SolarPanelValidationIcon.jpg')
  Voltage-Controlled Voltage Source - Scale panel voltage to Ns series panel : fl_lib/Electrical/Electrical Sources/Voltage-Controlled Voltage Source  K=-1*(solarPlant.numSeriesPanel-1)  v1_specify=off  v1_priority=None  v1=0 V  v1_nominal_specify=off  v1_nominal_value=1  v1_nominal_unit=V  v2_specify=off  v2_priority=None  v2=0 V  v2_nominal_specify=off  v2_nominal_value=1  v2_nominal_unit=V
  + : PMIOPort  Side=Right
  Irradiance : PMIOPort  Port=2  Side=Left
  - : PMIOPort  Port=3  Side=Right
  connections:
  Voltage-Controlled Voltage Source - Scale panel voltage to Ns series panel/RConn2 -- Voltage-Controlled Voltage Source - Scale panel voltage to Ns series panel/RConn1 -- Solar Panel/RConn1
  Voltage-Controlled Voltage Source - Scale panel voltage to Ns series panel/LConn1 -- Current-Controlled Current Source- Scale panel current to Np parallel strings/LConn2 -- -/RConn1 -- Solar Panel/RConn2
  Current-Controlled Current Source- Scale panel current to Np parallel strings/RConn1 -- Current-Controlled Current Source- Scale panel current to Np parallel strings/RConn2 -- +/RConn1
  Current-Controlled Current Source- Scale panel current to Np parallel strings/LConn1 -- Voltage-Controlled Voltage Source - Scale panel voltage to Ns series panel/LConn2
  Solar Panel/LConn1 -- Irradiance/RConn1

== system LunarMicrogrid_Combined_PVOnly_backup/BMS/DC Battery Current Sensor1 ==
  Current Sensor : fl_lib/Electrical/Electrical Sensors/Current Sensor
  PS-Simulink Converter : nesl_utility/PS-Simulink Converter  PhysicalDomain=network_engine_domain  SubClassName=ps_output  LeftPortType=input  RightPortType=output  PseudoPeriodic=off  Frequencies=[]  VectorFormat=1-D array  Unit=1  AffineConversion=off
  Sensor dynamics : TransferFcn  Numerator=1  Denominator=[1/sensor.samplingFreq 1]
  - : PMIOPort  Side=Left
  + : PMIOPort  Port=2  Side=Right
  tag scope: Ibattery=global
  wires:
  PS-Simulink Converter/1 -> Sensor dynamics/1
  Sensor dynamics/1 -> [Ibattery]
  connections:
  Current Sensor/RConn1 -- PS-Simulink Converter/LConn1
  +/RConn1 -- Current Sensor/LConn1
  Current Sensor/RConn2 -- -/RConn1

== system LunarMicrogrid_Combined_PVOnly_backup/BMS/DC Battery Voltage Sensor ==
  PS-Simulink Converter : nesl_utility/PS-Simulink Converter  PhysicalDomain=network_engine_domain  SubClassName=ps_output  LeftPortType=input  RightPortType=output  PseudoPeriodic=off  Frequencies=[]  VectorFormat=1-D array  Unit=1  AffineConversion=off
  Sensor dynamics : TransferFcn  Numerator=1  Denominator=[1/sensor.samplingFreq 1]
  Voltage Sensor : fl_lib/Electrical/Electrical Sensors/Voltage Sensor
      settings: LogSimulationData=on
  - : PMIOPort  Side=Left
  + : PMIOPort  Port=2  Side=Right
  tag scope: Vbat=global
  wires:
  PS-Simulink Converter/1 -> Sensor dynamics/1
  Sensor dynamics/1 -> [Vbat]
  connections:
  Voltage Sensor/LConn1 -- +/RConn1
  Voltage Sensor/RConn1 -- PS-Simulink Converter/LConn1
  Voltage Sensor/RConn2 -- -/RConn1

== system LunarMicrogrid_Combined_PVOnly_backup/Battery Management Control/Battery Charging ==
  note: Current controller
  note: Voltage Control
  Voref : Inport
  Vo : Inport  Port=2
  IL : Inport  Port=3
  Vbat : Inport  Port=4
  Enable : EnablePort  StatesWhenEnabling=reset
  Constant : Constant  Value=dcVoltage.reqDCBusVoltage
  Current control : Subsystem
  Divide : Product  Inputs=*/
  Saturation : Saturate  UpperLimit=1  LowerLimit=0
  Sum : Sum  Inputs=|+-
  Sum2 : Sum  Inputs=|--
  Sum3 : Sum  Inputs=|++
  Switch : Switch  Criteria=u2 > Threshold  Threshold=dcVoltage.reqDCBusVoltage*0.8  SaturateOnIntegerOverflow=off  InputSameDT=off
  Voltage control : Subsystem
  Mod : Outport
  wires:
  Voltage control/1(u) -> Sum2/1
  Voref/1 -> Switch/2, Switch/1, Sum/1
  Switch/1 -> Divide/2
  Sum2/1 -> Current control/1(e)
  Vo/1 -> Sum/2
  Current control/1(u) -> Sum3/1
  IL/1 -> Sum2/2
  Sum/1 -> Voltage control/1(e)
  Sum3/1 -> Saturation/1
  Saturation/1 -> Mod/1
  Constant/1 -> Switch/3
  Divide/1 -> Sum3/2
  Vbat/1 -> Divide/1

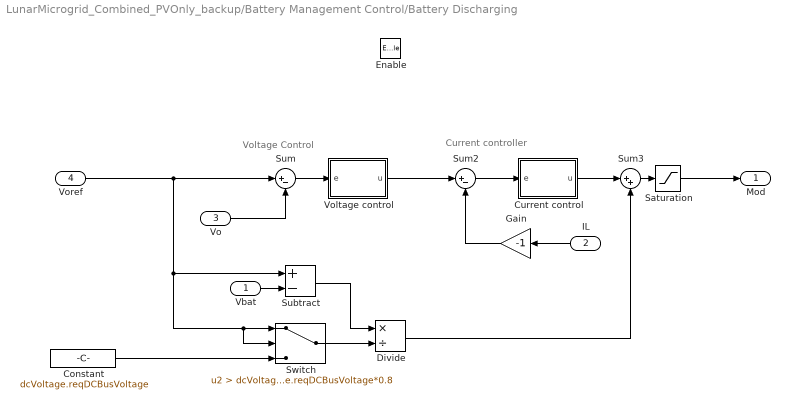
== system LunarMicrogrid_Combined_PVOnly_backup/Battery Management Control/Battery Discharging ==
  note: Current controller
  note: Voltage Control
  Vbat : Inport
  IL : Inport  Port=2
  Vo : Inport  Port=3
  Voref : Inport  Port=4
  Enable : EnablePort  StatesWhenEnabling=reset
  Constant : Constant  Value=dcVoltage.reqDCBusVoltage
  Current control : Subsystem
  Divide : Product  Inputs=*/
  Gain : Gain  Gain=-1
  Saturation : Saturate  UpperLimit=1  LowerLimit=0
  Subtract : Sum  Inputs=+-
  Sum : Sum  Inputs=|+-
  Sum2 : Sum  Inputs=|+-
  Sum3 : Sum  Inputs=|++
  Switch : Switch  Criteria=u2 > Threshold  Threshold=dcVoltage.reqDCBusVoltage*0.8  SaturateOnIntegerOverflow=off  InputSameDT=off
  Voltage control : Subsystem
  Mod : Outport
  wires:
  Voltage control/1(u) -> Sum2/1
  Voref/1 -> Sum/1, Subtract/1, Switch/2, Switch/1
  Switch/1 -> Divide/2
  Subtract/1 -> Divide/1
  Sum2/1 -> Current control/1(e)
  Vo/1 -> Sum/2
  Current control/1(u) -> Sum3/1
  IL/1 -> Gain/1
  Sum/1 -> Voltage control/1(e)
  Sum3/1 -> Saturation/1
  Saturation/1 -> Mod/1
  Vbat/1 -> Subtract/2
  Constant/1 -> Switch/3
  Gain/1 -> Sum2/2
  Divide/1 -> Sum3/2

== system LunarMicrogrid_Combined_PVOnly_backup/Battery Management Control/Charging ==
  mod : Inport
  Enable : EnablePort  StatesWhenEnabling=reset
  Constant : Constant  Value=0
  Gain : Gain
  Gain2 : Gain  Gain=5
  Rate Transition : RateTransition
  S1 : Outport
  S2 : Outport  Port=2
  wires:
  mod/1 -> Gain2/1
  Gain2/1 -> S1/1
  Constant/1 -> Gain/1
  Gain/1 -> Rate Transition/1
  Rate Transition/1 -> S2/1

== system LunarMicrogrid_Combined_PVOnly_backup/Battery Management Control/Discharging ==
  mod : Inport
  Enable : EnablePort  StatesWhenEnabling=reset
  Constant : Constant  Value=0
  Gain : Gain  Gain=5
  Gain1 : Gain
  Rate Transition : RateTransition
  S2 : Outport
  S1 : Outport  Port=2
  wires:
  mod/1 -> Gain/1
  Gain/1 -> S2/1
  Constant/1 -> Gain1/1
  Gain1/1 -> Rate Transition/1
  Rate Transition/1 -> S1/1

== system LunarMicrogrid_Combined_PVOnly_backup/Battery Management Control/Isolate ==
  Enable : EnablePort  StatesWhenEnabling=reset
  Constant : Constant  Value=0
  Constant1 : Constant  Value=0
  Gain : Gain
  Gain1 : Gain
  Rate Transition : RateTransition
  Rate Transition1 : RateTransition
  S2 : Outport
  S1 : Outport  Port=2
  wires:
  Constant/1 -> Gain/1
  Constant1/1 -> Gain1/1
  Gain/1 -> Rate Transition/1
  Gain1/1 -> Rate Transition1/1
  Rate Transition/1 -> S1/1
  Rate Transition1/1 -> S2/1

== system LunarMicrogrid_Combined_PVOnly_backup/Battery Management Control/PWM ==
  mod : Inport
  PWM Generator : eePwmGenerator/PWM Generator  CarrCount=Up  Tper=1/bms.batteryConverterSwitchingFrequency  Tdelay=0  Ts=1/(10*bms.batteryConverterSwitchingFrequency)
  Rate Transition1 : RateTransition  OutPortSampleTime=1/(10*bms.batteryConverterSwitchingFrequency)
  PWM : Outport
  wires:
  Rate Transition1/1 -> PWM Generator/1
  mod/1 -> Rate Transition1/1
  PWM Generator/1 -> PWM/1

== system LunarMicrogrid_Combined_PVOnly_backup/Boost Converter/AC Current Sensor1 ==
  Current Sensor : fl_lib/Electrical/Electrical Sensors/Current Sensor
  PS-Simulink Converter : nesl_utility/PS-Simulink Converter  PhysicalDomain=network_engine_domain  SubClassName=ps_output  LeftPortType=input  RightPortType=output  PseudoPeriodic=off  Frequencies=[]  VectorFormat=1-D array  Unit=1  AffineConversion=off
  Sensor dynamics : TransferFcn  Numerator=1  Denominator=[1/sensor.samplingFreq 1]
  - : PMIOPort  Side=Left
  + : PMIOPort  Port=2  Side=Right
  tag scope: IL=global
  wires:
  PS-Simulink Converter/1 -> Sensor dynamics/1
  Sensor dynamics/1 -> [IL]
  connections:
  Current Sensor/RConn1 -- PS-Simulink Converter/LConn1
  +/RConn1 -- Current Sensor/LConn1
  Current Sensor/RConn2 -- -/RConn1

== system LunarMicrogrid_Combined_PVOnly_backup/Load/AC Current Sensor2 ==
  Current Sensor : fl_lib/Electrical/Electrical Sensors/Current Sensor
  PS-Simulink Converter : nesl_utility/PS-Simulink Converter  PhysicalDomain=network_engine_domain  SubClassName=ps_output  LeftPortType=input  RightPortType=output  PseudoPeriodic=off  Frequencies=[]  VectorFormat=1-D array  Unit=1  AffineConversion=off
  Scope : Scope
      settings: ActiveDisplayYMinimum=-2.69141  ActiveDisplayYMaximum=24.19807  DataLoggingVariableName=ScopeData4
  Sensor dynamics : TransferFcn  Numerator=1  Denominator=[1/sensor.samplingFreq 1]
  - : PMIOPort  Side=Left
  + : PMIOPort  Port=2  Side=Right
  tag scope: Iload=global
  wires:
  PS-Simulink Converter/1 -> Sensor dynamics/1
  Sensor dynamics/1 -> Scope/1, [Iload]
  connections:
  Current Sensor/RConn1 -- PS-Simulink Converter/LConn1
  +/RConn1 -- Current Sensor/LConn1
  Current Sensor/RConn2 -- -/RConn1

== system LunarMicrogrid_Combined_PVOnly_backup/Load/Load ==
  " " : Constant
  " 1" : Constant  Value=1.5
  " 2" : Constant  Value=dcVoltage.reqDCBusVoltage*dcVoltage.reqDCBusVoltage*1e-3
  Divide : Product  Inputs=*/
  Load Power (kW) : Gain  Gain=lunarCase.P_kW
  Simulink-PS Converter1 : nesl_utility/Simulink-PS Converter  PhysicalDomain=network_engine_domain  SubClassName=ps_input  LeftPortType=input  RightPortType=output  PseudoPeriodic=off  Frequencies=[]  NoiseDistribution=none  NoiseParameters=[]  Unit=1  AffineConversion=off  FilteringAndDerivatives=provide  SimscapeFilterOrder=1  InputFilterTimeConstant=0.001  UdotUserProvided=0
  Switch : Switch  Criteria=u2 > Threshold  SaturateOnIntegerOverflow=off  InputSameDT=off
  R : PMIOPort  Side=Right
  wires:
  " "/1 -> Load Power (kW)/1
  Load Power (kW)/1 -> Switch/1, Switch/2
  " 1"/1 -> Switch/3
  " 2"/1 -> Divide/1
  Switch/1 -> Divide/2
  Divide/1 -> Simulink-PS Converter1/1
  connections:
  Simulink-PS Converter1/RConn1 -- R/RConn1

== system LunarMicrogrid_Combined_PVOnly_backup/Load/Load Flag ==
  Data Type Conversion1 : DataTypeConversion  SaturateOnIntegerOverflow=off  RndMeth=Floor
  NOT : Logic  Operator=NOT  IconShape=distinctive  AllPortsSameDT=off  OutDataTypeStr=boolean
  OR : Logic  Operator=OR  IconShape=distinctive  AllPortsSameDT=off  OutDataTypeStr=boolean
  Simulink-PS Converter2 : nesl_utility/Simulink-PS Converter  PhysicalDomain=network_engine_domain  SubClassName=ps_input  LeftPortType=input  RightPortType=output  PseudoPeriodic=off  Frequencies=[]  NoiseDistribution=none  NoiseParameters=[]  Unit=1  AffineConversion=off  FilteringAndDerivatives=provide  SimscapeFilterOrder=1  InputFilterTimeConstant=0.001  UdotUserProvided=0
  CB : PMIOPort  Side=Right
  wires:
  [loadShutDown] -> OR/1
  Data Type Conversion1/1 -> Simulink-PS Converter2/1
  [ShutDown] -> OR/2  "System Status"
  OR/1 -> NOT/1
  NOT/1 -> Data Type Conversion1/1
  connections:
  Simulink-PS Converter2/RConn1 -- CB/RConn1

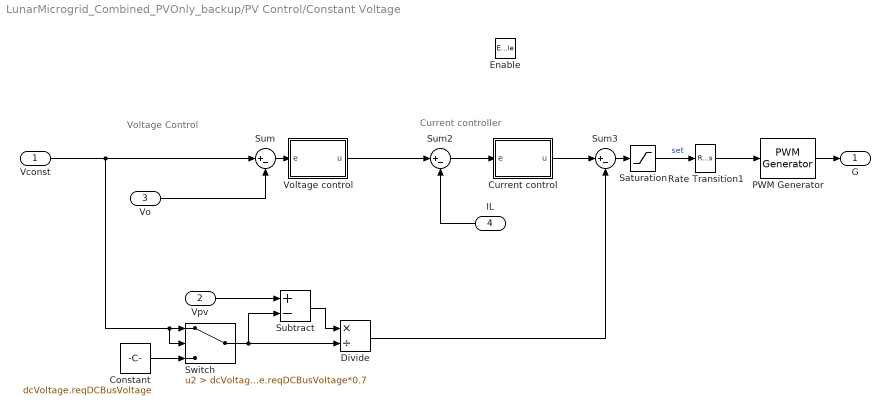
== system LunarMicrogrid_Combined_PVOnly_backup/PV Control/Constant Voltage ==
  note: Current controller
  note: Voltage Control
  Vconst : Inport
  Vpv : Inport  Port=2
  "Vo " : Inport  Port=3
  IL : Inport  Port=4
  Enable : EnablePort  StatesWhenEnabling=reset
  Constant : Constant  Value=dcVoltage.reqDCBusVoltage
  Current control : Subsystem
  Divide : Product  Inputs=*/
  PWM Generator : eePwmGenerator/PWM Generator  CarrCount=Up  Tper=1/solarPlant.converterSwitchingFrequency  Tdelay=0  Ts=1/(10*solarPlant.converterSwitchingFrequency)
  Rate Transition1 : RateTransition  OutPortSampleTime=1/(10*solarPlant.converterSwitchingFrequency)
  Saturation : Saturate  UpperLimit=1  LowerLimit=0
  Subtract : Sum  Inputs=+-
  Sum : Sum  Inputs=|+-
  Sum2 : Sum  Inputs=|+-
  Sum3 : Sum  Inputs=|+-
  Switch : Switch  Criteria=u2 > Threshold  Threshold=dcVoltage.reqDCBusVoltage*0.7  SaturateOnIntegerOverflow=off  InputSameDT=off
  Voltage control : Subsystem
  G : Outport
  wires:
  Switch/1 -> Divide/2, Subtract/2
  Constant/1 -> Switch/3
  "Vo "/1 -> Sum/2
  Vconst/1 -> Switch/2, Switch/1, Sum/1
  Divide/1 -> Sum3/2
  PWM Generator/1 -> G/1
  Rate Transition1/1 -> PWM Generator/1
  Sum3/1 -> Saturation/1
  Vpv/1 -> Subtract/1
  Sum/1 -> Voltage control/1(e)
  Voltage control/1(u) -> Sum2/1
  Current control/1(u) -> Sum3/1
  Sum2/1 -> Current control/1(e)
  Subtract/1 -> Divide/1
  Saturation/1 -> Rate Transition1/1  "set"
  IL/1 -> Sum2/2
